simulink model "boost_simulink"  (R2024a)
settings: Solver=VariableStepAuto  StartTime=0.0  StopTime=15  FixedStep=0.01  RelTol=1e-3
StopFcn:
  | boostIO('stop'); pause(0.1); clear boostIO
values from neighbouring files (symbols this model uses):
  Ki = Ki_all(dBest)    [Run_HW_PI_Optimization.m]    (also in Run_PI_Hardware_Optimization.m = Ki_all(ord(1)); Run_PI_Hardware_Optimization_1.m; run_boost_test.m = 20)
  Kp = Kp_all(dBest)    [Run_HW_PI_Optimization.m]    (also in Run_PI_Hardware_Optimization.m = Kp_all(ord(1)); Run_PI_Hardware_Optimization_1.m; run_boost_test.m = 0.1)
  t_step = 3    [run_boost_test.m]    (also in tune_boost_kpki.m = 2)
  V0 = 8    [run_boost_test.m]    (also in tune_boost_kpki.m)
  V1 = 15    [run_boost_test.m]    (also in tune_boost_kpki.m = 12)
settings Model: Creator=Razowan  LastModifiedBy=Razowan

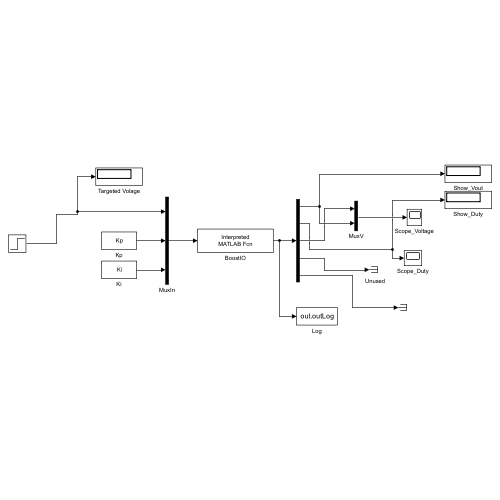
[thumbnail: Simulink's stored preview of the top-level diagram]
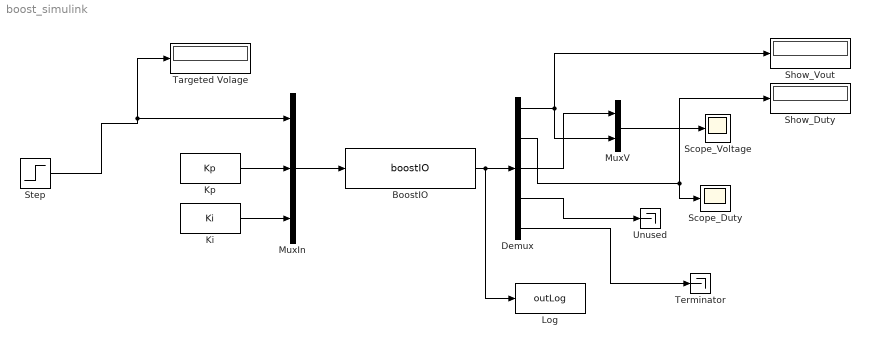
== system boost_simulink ==
  BoostIO : MATLABFcn  MATLABFcn=boostIO  OutputDimensions=5  OutputSignalType=real  SampleTime=0.01
  Demux : Demux  Outputs=5
  Ki : Constant  Value=Ki
  Kp : Constant  Value=Kp
  Log : ToWorkspace  VariableName=outLog  SampleTime=-1
  MuxIn : Mux  Inputs=3
  MuxV : Mux  Inputs=2
  Scope_Duty : Scope
  Scope_Voltage : Scope
  Show_Duty : Display
  Show_Vout : Display
  Step : Step  Time=t_step  Before=V0  After=V1  SampleTime=.01
  Targeted Volage : Display
  Terminator : Terminator
  Unused : Terminator
  wires:
  Step/1 -> Targeted Volage/1, MuxIn/1
  Kp/1 -> MuxIn/2
  Ki/1 -> MuxIn/3
  MuxIn/1 -> BoostIO/1
  BoostIO/1 -> Log/1, Demux/1
  Demux/3 -> MuxV/1
  Demux/1 -> MuxV/2, Show_Vout/1
  MuxV/1 -> Scope_Voltage/1
  Demux/2 -> Scope_Duty/1, Show_Duty/1
  Demux/4 -> Unused/1
  Demux/5 -> Terminator/1
